simulink model "Pendulum_Simulink"  (R2026b)
settings: Solver=VariableStepAuto  StopTime=30
InitFcn:
  | InvertedPendulum
values from neighbouring files (symbols this model uses):
  G0_den = [1 b -K]    [InvertedPendulum.m]
  G0_num = [0 0 c]    [InvertedPendulum.m]
  ImpulseMag = 30    [InvertedPendulum.m]
  w_car = pi/3    (= 1.0471975512)    [InvertedPendulum.m]
undefined symbols (not defined in the file or in its folder): C_den, C_num
libraries: simulink x2
settings Model: Creator=slaga  LastModifiedBy=slaga

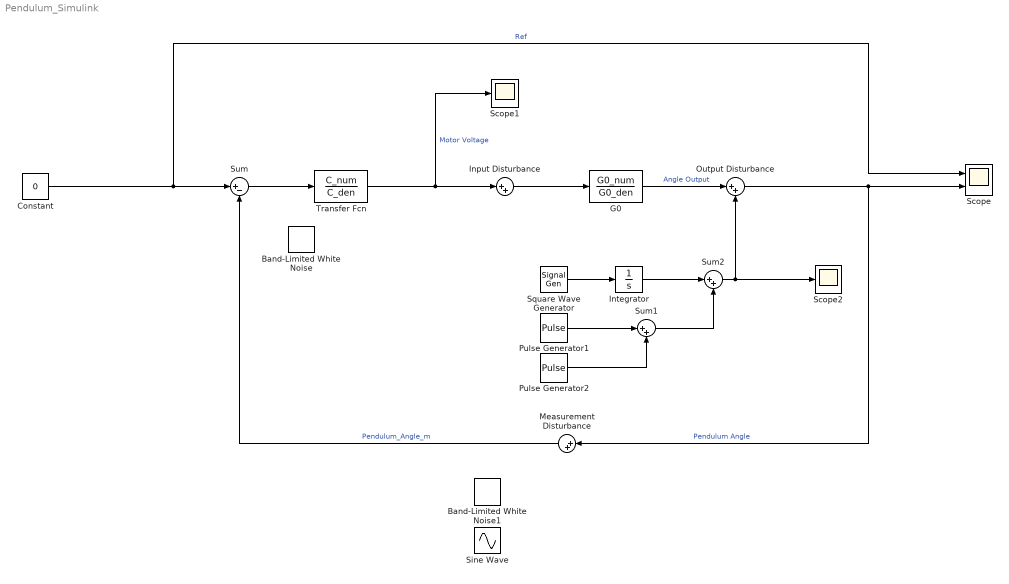
== system Pendulum_Simulink ==
  Band-Limited White Noise : simulink/Sources/Band-Limited White Noise  Cov=[0.01]  Ts=0.1  seed=[23341]
  Band-Limited White Noise1 : simulink/Sources/Band-Limited White Noise  Cov=[0.01]  Ts=0.1  seed=[23341]
  Constant : Constant  Value=0
  G0 : TransferFcn  Numerator=G0_num  Denominator=G0_den
  Input Disturbance : Sum  Inputs=|++
  Integrator : Integrator
  Measurement Disturbance : Sum  Inputs=|++
  Output Disturbance : Sum  Inputs=|++
  Pulse Generator1 : DiscretePulseGenerator  PulseType=Time based  Amplitude=(pi/180)*ImpulseMag  Period=6  PulseWidth=0.1  PhaseDelay=3
  Pulse Generator2 : DiscretePulseGenerator  PulseType=Time based  Amplitude=-(pi/180)*ImpulseMag  Period=6  PulseWidth=0.1
  Scope : Scope  NumInputPorts=2
      settings: ActiveDisplayYMinimum=-1.0038855012430652  ActiveDisplayYMaximum=1.0855709894702263
  Scope1 : Scope
      settings: ActiveDisplayYMinimum=-42.237501232876077  ActiveDisplayYMaximum=40.067584277200289
  Scope2 : Scope
      settings: ActiveDisplayYMinimum=-7.042877821190844  ActiveDisplayYMaximum=0.76857934611640233  DataLoggingVariableName=ScopeData2
  Sine Wave : Sin  Amplitude=0.1  Frequency=100  SampleTime=0
  Square Wave Generator : SignalGenerator  WaveForm=square  Amplitude=w_car  Frequency=1/6
  Sum : Sum  Inputs=|+-
  Sum1 : Sum  Inputs=|++
  Sum2 : Sum  Inputs=|++
  Transfer Fcn : TransferFcn  Numerator=C_num  Denominator=C_den
  wires:
  Sum/1 -> Transfer Fcn/1
  Constant/1 -> Scope/1, Sum/1  "Ref"
  G0/1 -> Output Disturbance/1  "Angle Output"
  Output Disturbance/1 -> Measurement Disturbance/1, Scope/2  "Pendulum Angle"
  Input Disturbance/1 -> G0/1
  Transfer Fcn/1 -> Scope1/1, Input Disturbance/1  "Motor Voltage"
  Measurement Disturbance/1 -> Sum/2  "Pendulum_Angle_m"
  Square Wave Generator/1 -> Integrator/1
  Pulse Generator1/1 -> Sum1/1
  Pulse Generator2/1 -> Sum1/2
  Integrator/1 -> Sum2/1
  Sum1/1 -> Sum2/2
  Sum2/1 -> Scope2/1, Output Disturbance/2
